simulink model "ins01"  (Simulink 4.00)
settings: Solver=ode45  StartTime=0.0  StopTime=5040  RelTol=1e-3
values from neighbouring files (symbols this model uses):
  A = [0,                     0,  1/R,    0,          0,  0,  0,  Vn/R^2,         0 ... (first row only)    [Ainit.m]    (also in build17StateSysDyn.m = Rot'*[An; Ae]; build28StateTransMat.m = Rot'*[An; Ae])
  B = zeros(9,9)    [Ainit.m]
  C = eye(9)    [Ainit.m]
  D = zeros(9,9)    [Ainit.m]    (also in compute_ud.m = [])
  rad2mrad = 10e6    (= 10000000)    [Ainit.m]
  x0 = [lat,lon,Vn,Ve,0,0,0,-R,0]'    [Ainit.m]
settings Model: Creator=mcar  LastModifiedBy=mcar  BlockReductionOpt=off

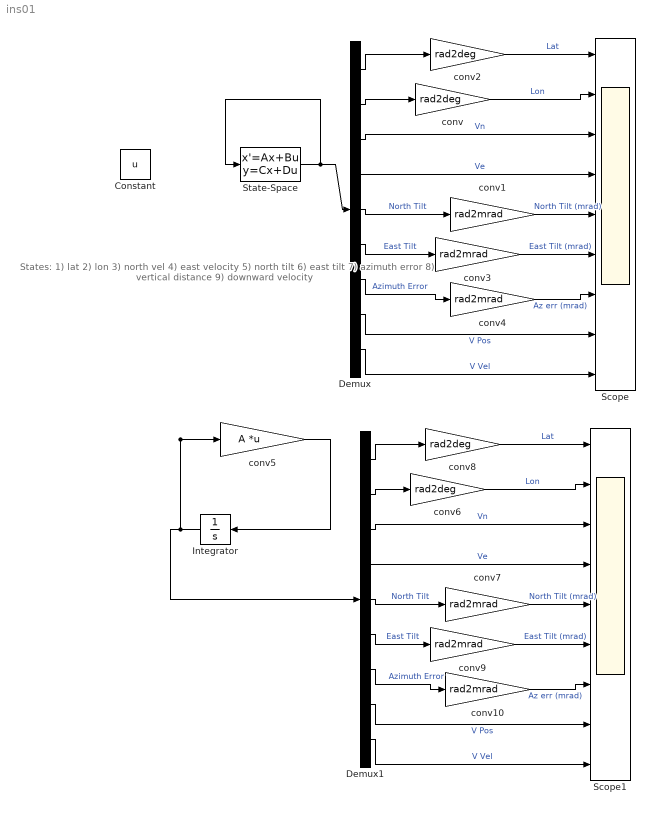
== system ins01 ==
  note: States:
      | 1) lat
      | 2) lon
      | 3) north vel
      | 4) east velocity
      | 5) north tilt
      | 6) east tilt
      | 7) azimuth error
      | 8) vertical distance
      | 9) downward velocity
  Constant : Constant  Value=u
  Demux : Demux  Outputs=9  BusSelectionMode=off
  Demux1 : Demux  Outputs=9  BusSelectionMode=off
  Integrator : Integrator  Orientation=left  ExternalReset=none  InitialConditionSource=internal  InitialCondition=x0  LimitOutput=off  UpperSaturationLimit=inf  LowerSaturationLimit=-inf  ShowSaturationPort=off  ShowStatePort=off  AbsoluteTolerance=auto
  Scope : Scope  NumInputPorts=9
      settings: TimeRange=auto  YMin=-5~-5~-5~-5~-5~-5~-5~-5~-5  YMax=5~5~5~5~5~5~5~5~5  SaveToWorkspace=off  SaveName=ScopeData  LimitDataPoints=on  MaxDataPoints=5000
  Scope1 : Scope  NumInputPorts=9
      settings: TimeRange=6000  YMin=-500~-20000~0~-5000000~0~-100000000~-2000000000~-40000000000~-40000000  YMax=500~0~40000~5000000~4000000000~100000000~2000000000~0~0  SaveToWorkspace=off  LimitDataPoints=on  MaxDataPoints=5000
  State-Space : StateSpace  A=A  B=B  C=C  D=D  X0=x0  Realization=auto  AbsoluteTolerance=auto
  conv{,2,6,8} (4 alike) : Gain  Gain=rad2deg  Multiplication=Element-wise(K.*u)  SaturateOnIntegerOverflow=on
  conv{1,3..4,7,9..10} (6 alike) : Gain  Gain=rad2mrad  Multiplication=Element-wise(K.*u)  SaturateOnIntegerOverflow=on
  conv5 : Gain  Gain=A  Multiplication=Matrix(K*u)  SaturateOnIntegerOverflow=on
  wires:
  State-Space/1 -> Demux/1, State-Space/1
  Demux/1 -> conv2/1
  Demux/2 -> conv/1
  Demux/3 -> Scope/3  "Vn"
  Demux/4 -> Scope/4  "Ve"
  Demux/5 -> conv1/1  "North Tilt"
  Demux/6 -> conv3/1  "East Tilt"
  Demux/7 -> conv4/1  "Azimuth Error"
  Demux/8 -> Scope/8  "V Pos"
  Demux/9 -> Scope/9  "V Vel"
  conv2/1 -> Scope/1  "Lat"
  conv/1 -> Scope/2  "Lon"
  conv1/1 -> Scope/5  "North Tilt (mrad)"
  conv3/1 -> Scope/6  "East Tilt (mrad)"
  conv4/1 -> Scope/7  "Az err (mrad)"
  Demux1/1 -> conv8/1
  Demux1/2 -> conv6/1
  Demux1/3 -> Scope1/3  "Vn"
  Demux1/4 -> Scope1/4  "Ve"
  Demux1/5 -> conv7/1  "North Tilt"
  Demux1/6 -> conv9/1  "East Tilt"
  Demux1/7 -> conv10/1  "Azimuth Error"
  Demux1/8 -> Scope1/8  "V Pos"
  Demux1/9 -> Scope1/9  "V Vel"
  conv8/1 -> Scope1/1  "Lat"
  conv6/1 -> Scope1/2  "Lon"
  conv7/1 -> Scope1/5  "North Tilt (mrad)"
  conv9/1 -> Scope1/6  "East Tilt (mrad)"
  conv10/1 -> Scope1/7  "Az err (mrad)"
  conv5/1 -> Integrator/1
  Integrator/1 -> Demux1/1, conv5/1
